simulink model "model"  (R2024b)
settings: Solver=VariableStepAuto  StartTime=0.0  StopTime=25  RelTol=1e-3
PreLoadFcn:
  | StartupProject;
  | createVariables;
undefined symbols (not defined in the file or in its folder): diff, eour6dof, Levenberg, Marquardt, maxWaypoints, ts, waypointTimes, X, Y, Z
libraries: sm_lib x46, nesl_utility x13, blocksLibrary x8, robotcorelib x3, robotmaniplib x1
(part 2 of 2)

== system model/Plant/Arm/link_7 ==
  Reference Frame : sm_lib/Frames and Transforms/Reference Frame
  link_7 : sm_lib/Body Elements/File Solid  ExtGeomFileName=./meshes/link_7.stl  UnitType=Custom  ExtGeomFileUnits=mm  StepReaderType=HEX  ExportConvexHullGeometry=off  InertiaType=CalculateFromGeometry  BasedOnType=Mass  Density=7986.89  DensityUnits=kg/m^3  Mass=680.695  MassUnits=g  CenterOfMass=[0.00, 0.00, 7.613]  CenterOfMassUnits=mm  MomentsOfInertia=[1 1 1]  MomentsOfInertiaUnits=g*mm^2  ProductsOfInertia=[0 0 0]  ProductsOfInertiaUnits=g*mm^2  GraphicType=FromGeometry  MarkerShape=Sphere  MarkerSize=10  GraphicVisPropType=SimpleVisualProperties  GraphicDiffuseColor=[0.5 0.5 0.5]  GraphicOpacity=1.0  GraphicSpecularColor=[0.5 0.5 0.5 1.0]  GraphicAmbientColor=[0.15 0.15 0.15 1.0]  GraphicEmissiveColor=[0.0 0.0 0.0 1.0]  GraphicShininess=75  DoExposeReferenceFrame=on  SerializedFrames=<Frames/>
  joint 6 : PMIOPort  Side=Left
  connections:
  joint 6/RConn1 -- Reference Frame/RConn1 -- link_7/RConn1
